simulink model "whrobot"  (R2022a)
settings: Solver=VariableStepAuto  StartTime=0.0  StopTime=30  RelTol=1e-6
undefined symbols (not defined in the file or in its folder): D, dt, h, L, m, theta0, v0, w, w0, x0, y0
libraries: rllib x1
settings Model: Creator=mtearle
settings SolverCC: AlgebraicLoopSolver=TrustRegion
settings DebuggingCC: UnconnectedInputMsg=warning  UnconnectedOutputMsg=warning  UnconnectedLineMsg=warning

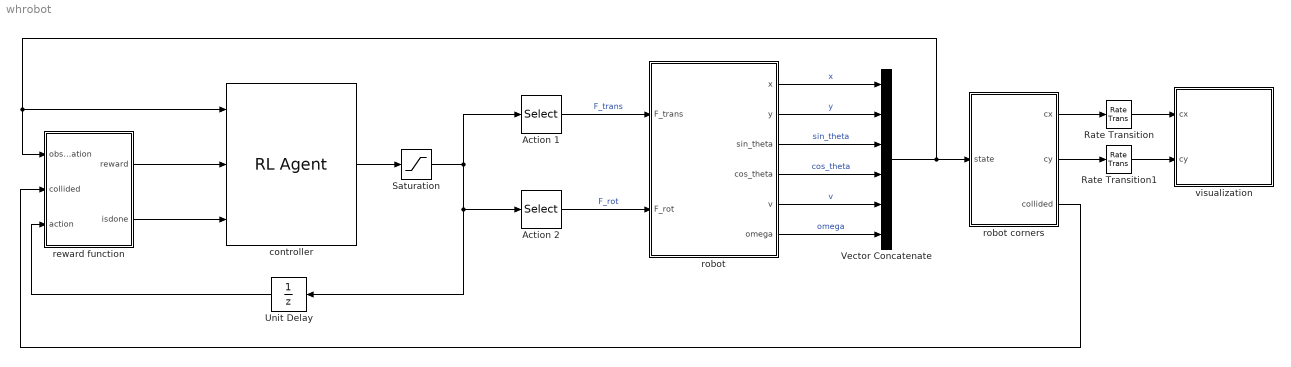
== system whrobot ==
  Action 1 : Selector  InputPortWidth=2  IndexOptions=Index vector (dialog)  Indices=1  OutputSizes=1
  Action 2 : Selector  InputPortWidth=2  IndexOptions=Index vector (dialog)  Indices=2  OutputSizes=1
  Rate Transition : RateTransition  OutPortSampleTime=dt
  Rate Transition1 : RateTransition  OutPortSampleTime=dt
  Saturation : Saturate  UpperLimit=1  LowerLimit=-1
  Unit Delay : UnitDelay  SampleTime=-1  HasFrameUpgradeWarning=on
  Vector Concatenate : Concatenate  NumInputs=6
  controller : rllib/RL Agent  Agent=agent  ExternalActionAsInput=off  ProvideLastAction=off  ProvideCumRwd=off  TreatAsDirectFeedthrough=on  UseStrictObservationDataTypes=off
  reward function : MATLAB Function  TreatAsAtomicUnit=on
  robot : Subsystem  SystemSampleTime=0.1
  robot corners : MATLAB Function  TreatAsAtomicUnit=on
  visualization : MATLAB Function  TreatAsAtomicUnit=on
  wires:
  robot/3(sin_theta) -> Vector Concatenate/3  "sin_theta"
  robot/4(cos_theta) -> Vector Concatenate/4  "cos_theta"
  Action 2/1 -> robot/2(F_rot)  "F_rot"
  Action 1/1 -> robot/1(F_trans)  "F_trans"
  Rate Transition/1 -> visualization/1(cx)
  Unit Delay/1 -> reward function/3(action)
  controller/1 -> Saturation/1
  robot/1(x) -> Vector Concatenate/1  "x"
  reward function/1(reward) -> controller/2
  reward function/2(isdone) -> controller/3
  robot/2(y) -> Vector Concatenate/2  "y"
  Saturation/1 -> Action 2/1, Unit Delay/1, Action 1/1
  robot/5(v) -> Vector Concatenate/5  "v"
  robot/6(omega) -> Vector Concatenate/6  "omega"
  robot corners/1(cx) -> Rate Transition/1
  Rate Transition1/1 -> visualization/2(cy)
  robot corners/2(cy) -> Rate Transition1/1
  robot corners/3(collided) -> reward function/2(collided)
  Vector Concatenate/1 -> controller/1, reward function/1(observation), robot corners/1(state)

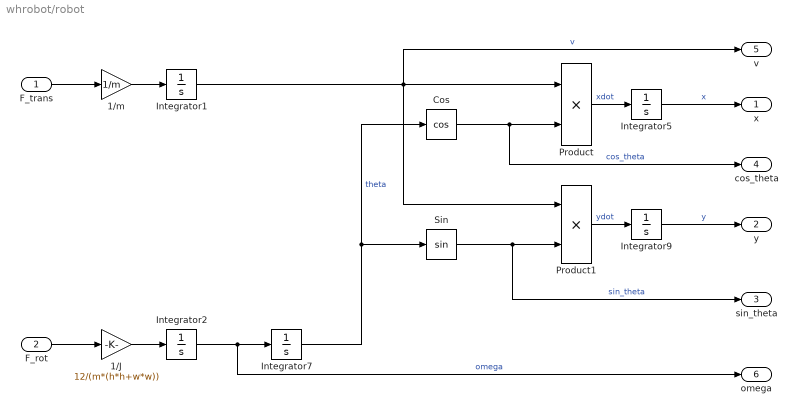
== system whrobot/robot ==
  F_trans : Inport
  F_rot : Inport  Port=2
  1/J : Gain  Gain=12/(m*(h*h+w*w))
  1/m : Gain  Gain=1/m
  Cos : Trigonometry  Operator=cos
  Integrator1 : Integrator  InitialCondition=v0  LimitOutput=on  UpperSaturationLimit=5  LowerSaturationLimit=-5
  Integrator2 : Integrator  InitialCondition=w0  LimitOutput=on  UpperSaturationLimit=2*pi  LowerSaturationLimit=-2*pi
  Integrator5 : Integrator  InitialCondition=x0
  Integrator7 : Integrator  InitialCondition=theta0  UpperSaturationLimit=pi/2  WrapState=on
  Integrator9 : Integrator  InitialCondition=y0
  Product : Product
  Product1 : Product
  Sin : Trigonometry
  x : Outport  SampleTime=dt
  y : Outport  Port=2  SampleTime=dt
  sin_theta : Outport  Port=3  SampleTime=dt
  cos_theta : Outport  Port=4  SampleTime=dt
  v : Outport  Port=5  SampleTime=dt
  omega : Outport  Port=6
  wires:
  Product1/1 -> Integrator9/1  "ydot"
  Integrator7/1 -> Cos/1, Sin/1  "theta"
  F_trans/1 -> 1/m/1
  Sin/1 -> sin_theta/1, Product1/2  "sin_theta"
  Product/1 -> Integrator5/1  "xdot"
  Cos/1 -> cos_theta/1, Product/2  "cos_theta"
  Integrator9/1 -> y/1  "y"
  Integrator5/1 -> x/1  "x"
  F_rot/1 -> 1/J/1
  Integrator1/1 -> v/1, Product1/1, Product/1  "v"
  Integrator2/1 -> omega/1, Integrator7/1  "omega"
  1/m/1 -> Integrator1/1
  1/J/1 -> Integrator2/1

== matlab function whrobot/robot corners ==
  data: state input; cx output; cy output; h parameter; w parameter; collided output; L parameter; D parameter
function [cx,cy,collided] = getcorners(state,h,w,L, D)

% preallocate outputs
% cx = zeros(4,1);
% cy = zeros(4,1);

% extract individual components
x = state(1);
y = state(2);
s = state(3);
c = state(4);

% four corners
p = [h,-h,-h,h;w,w,-w,-w]/2;

% rotation matrix
M = [c,-s;s,c];

% rotate points
p = M*p;
% translate and extract x,y
cx = x*ones(1,4) + p(1,:);
cy = y*ones(1,4) + p(2,:);

% bottom obstacles
% corners of obstacle inside the robot (corner sideswipe)
collided = any(inpolygon([-L;L],[D;D],cx,cy));
% corner of robot inside obstacle(hit obstacle)
collided = collided || any((cy < D) & (abs(cx) > L));
% vertical obstacle
% corners of obstacle inside the robot (corner sideswipe)
collided = collided || any(inpolygon([-L;L],3*[D;D],cx,cy));
% corner of robot inside obstacle(hit obstacle)
collided = collided || any((cy > 3*D) & (abs(cx) < L));

== matlab function whrobot/reward function ==
  data: observation input; collided input; action input; reward output; isdone output
function [reward,isdone] = reward(observation, collided, action)

% out through the bottom?
y = observation(2);
madeit = (y < -1.5);

% calculate reward value
reward = rewardfun(observation,action,madeit,collided);

% done if either failed (crashed) or succeeded
isdone = collided || madeit;

== matlab function whrobot/visualization ==
  data: cx input; cy input; D parameter; L parameter
function drawEnvironment(cx,cy,D,L)

coder.extrinsic("plotRobot");
plotRobot(cx,cy,D,L);
